simulink model "mano_buena_pinza_paper"  (R2025a)
settings: Solver=ode23  StartTime=0.0  StopTime=10.5  FixedStep=20e-3  MaxStep=1e-3  RelTol=1e-2  AbsTol=1e-4
model workspace: external: MATLAB File mano_vf_DataFile1.m (data not in the file)
undefined symbols (not defined in the file): smiData, X, Y, Z
libraries: sm_lib x268, nesl_utility x26
(part 7 of 7)

== system mano_buena_pinza_paper/Pulgar/Pulgar4/Tierra_pulgar1_RIGID ==
  ReferenceFrame : sm_lib/Frames and Transforms/Reference Frame
  Solid : sm_lib/Body Elements/File Solid  ExtGeomFileName=Tierra_pulgar_ipt_749dbfaf.STEP  UnitType=FromFile  ExtGeomFileUnits=m  StepReaderType=HEX  ExportConvexHullGeometry=on  InertiaType=Custom  BasedOnType=DensityFromFile  Density=1000  DensityUnits=kg/m^3  Mass=smiData.Solid(3).mass  MassUnits=kg  CenterOfMass=smiData.Solid(3).CoM  CenterOfMassUnits=mm  MomentsOfInertia=smiData.Solid(3).MoI  MomentsOfInertiaUnits=kg*mm^2  ProductsOfInertia=smiData.Solid(3).PoI  ProductsOfInertiaUnits=kg*mm^2  GraphicType=FromGeometry  MarkerShape=Sphere  MarkerSize=10  GraphicVisPropType=SimpleVisualProperties  GraphicDiffuseColor=smiData.Solid(3).color  GraphicOpacity=smiData.Solid(3).opacity  GraphicSpecularColor=[0.5 0.5 0.5 1.0]  GraphicAmbientColor=[0.15 0.15 0.15 1.0]  GraphicEmissiveColor=[0.0 0.0 0.0 1.0]  GraphicShininess=75  DoExposeReferenceFrame=on  SerializedFrames=<Frames/>
  Transform : sm_lib/Frames and Transforms/Rigid Transform  RotationMethod=ArbitraryAxis  FollAlignAxisA=+X  BaseAlignAxisA=+Y  FollAlignAxisB=+Y  BaseAlignAxisB=+Z  RotationStandardAxis=+Z  RotationAngle=smiData.RigidTransform(82).angle  RotationAngleUnits=rad  RotationArbitraryAxis=smiData.RigidTransform(82).axis  RotationSequenceAxes=FollowerAxes  RotationSequence=XYX  RotationSequenceAngles=[0 0 0]  RotationSequenceAnglesUnits=deg  RotationMatrix=[1 0 0;0 1 0;0 0 1]  Quaternion=[1 0 0 0]  TranslationMethod=Cartesian  TranslationCartesianOffset=smiData.RigidTransform(82).translation  TranslationCartesianOffsetUnits=mm  TranslationStandardAxis=+Z  TranslationStandardOffset=0  TranslationStandardOffsetUnits=m  TranslationROffset=0  TranslationROffsetUnits=m  TranslationThetaOffset=0  TranslationThetaOffsetUnits=deg  TranslationZOffset=0  TranslationZOffsetUnits=m
  Transform1 : sm_lib/Frames and Transforms/Rigid Transform  RotationMethod=ArbitraryAxis  FollAlignAxisA=+X  BaseAlignAxisA=+Y  FollAlignAxisB=+Y  BaseAlignAxisB=+Z  RotationStandardAxis=+Z  RotationAngle=smiData.RigidTransform(91).angle  RotationAngleUnits=rad  RotationArbitraryAxis=smiData.RigidTransform(91).axis  RotationSequenceAxes=FollowerAxes  RotationSequence=XYX  RotationSequenceAngles=[0 0 0]  RotationSequenceAnglesUnits=deg  RotationMatrix=[1 0 0;0 1 0;0 0 1]  Quaternion=[1 0 0 0]  TranslationMethod=Cartesian  TranslationCartesianOffset=smiData.RigidTransform(91).translation  TranslationCartesianOffsetUnits=mm  TranslationStandardAxis=+Z  TranslationStandardOffset=0  TranslationStandardOffsetUnits=m  TranslationROffset=0  TranslationROffsetUnits=m  TranslationThetaOffset=0  TranslationThetaOffsetUnits=deg  TranslationZOffset=0  TranslationZOffsetUnits=m
  F : PMIOPort  Side=Left
  F1 : PMIOPort  Port=2  Side=Right
  F2 : PMIOPort  Port=3  Side=Right
  connections:
  Solid/RConn1 -- ReferenceFrame/RConn1 -- Transform/LConn1 -- Transform1/LConn1
  Transform/RConn1 -- F/RConn1
  Transform1/RConn1 -- F1/RConn1
  F2/RConn1 -- Solid/LConn1

== system mano_buena_pinza_paper/Pulgar/Pulgar4/distal_pulgar1_RIGID ==
  ReferenceFrame : sm_lib/Frames and Transforms/Reference Frame
  Solid : sm_lib/Body Elements/File Solid  ExtGeomFileName=distal_pulgar_ipt_baa67ac8.STEP  UnitType=FromFile  ExtGeomFileUnits=m  StepReaderType=HEX  ExportConvexHullGeometry=on  InertiaType=Custom  BasedOnType=DensityFromFile  Density=1000  DensityUnits=kg/m^3  Mass=smiData.Solid(5).mass  MassUnits=kg  CenterOfMass=smiData.Solid(5).CoM  CenterOfMassUnits=mm  MomentsOfInertia=smiData.Solid(5).MoI  MomentsOfInertiaUnits=kg*mm^2  ProductsOfInertia=smiData.Solid(5).PoI  ProductsOfInertiaUnits=kg*mm^2  GraphicType=FromGeometry  MarkerShape=Sphere  MarkerSize=10  GraphicVisPropType=SimpleVisualProperties  GraphicDiffuseColor=smiData.Solid(5).color  GraphicOpacity=smiData.Solid(5).opacity  GraphicSpecularColor=[0.5 0.5 0.5 1.0]  GraphicAmbientColor=[0.15 0.15 0.15 1.0]  GraphicEmissiveColor=[0.0 0.0 0.0 1.0]  GraphicShininess=75  DoExposeReferenceFrame=on  SerializedFrames=<Frames/>
  Transform : sm_lib/Frames and Transforms/Rigid Transform  RotationMethod=ArbitraryAxis  FollAlignAxisA=+X  BaseAlignAxisA=+Y  FollAlignAxisB=+Y  BaseAlignAxisB=+Z  RotationStandardAxis=+Z  RotationAngle=smiData.RigidTransform(35).angle  RotationAngleUnits=rad  RotationArbitraryAxis=smiData.RigidTransform(35).axis  RotationSequenceAxes=FollowerAxes  RotationSequence=XYX  RotationSequenceAngles=[0 0 0]  RotationSequenceAnglesUnits=deg  RotationMatrix=[1 0 0;0 1 0;0 0 1]  Quaternion=[1 0 0 0]  TranslationMethod=Cartesian  TranslationCartesianOffset=smiData.RigidTransform(35).translation  TranslationCartesianOffsetUnits=mm  TranslationStandardAxis=+Z  TranslationStandardOffset=0  TranslationStandardOffsetUnits=m  TranslationROffset=0  TranslationROffsetUnits=m  TranslationThetaOffset=0  TranslationThetaOffsetUnits=deg  TranslationZOffset=0  TranslationZOffsetUnits=m
  Transform1 : sm_lib/Frames and Transforms/Rigid Transform  RotationMethod=ArbitraryAxis  FollAlignAxisA=+X  BaseAlignAxisA=+Y  FollAlignAxisB=+Y  BaseAlignAxisB=+Z  RotationStandardAxis=+Z  RotationAngle=smiData.RigidTransform(39).angle  RotationAngleUnits=rad  RotationArbitraryAxis=smiData.RigidTransform(39).axis  RotationSequenceAxes=FollowerAxes  RotationSequence=XYX  RotationSequenceAngles=[0 0 0]  RotationSequenceAnglesUnits=deg  RotationMatrix=[1 0 0;0 1 0;0 0 1]  Quaternion=[1 0 0 0]  TranslationMethod=Cartesian  TranslationCartesianOffset=smiData.RigidTransform(39).translation  TranslationCartesianOffsetUnits=mm  TranslationStandardAxis=+Z  TranslationStandardOffset=0  TranslationStandardOffsetUnits=m  TranslationROffset=0  TranslationROffsetUnits=m  TranslationThetaOffset=0  TranslationThetaOffsetUnits=deg  TranslationZOffset=0  TranslationZOffsetUnits=m
  Transform2 : sm_lib/Frames and Transforms/Rigid Transform  RotationMethod=ArbitraryAxis  FollAlignAxisA=+X  BaseAlignAxisA=+Y  FollAlignAxisB=+Y  BaseAlignAxisB=+Z  RotationStandardAxis=+Z  RotationAngle=smiData.RigidTransform(92).angle  RotationAngleUnits=rad  RotationArbitraryAxis=smiData.RigidTransform(92).axis  RotationSequenceAxes=FollowerAxes  RotationSequence=XYX  RotationSequenceAngles=[0 0 0]  RotationSequenceAnglesUnits=deg  RotationMatrix=[1 0 0;0 1 0;0 0 1]  Quaternion=[1 0 0 0]  TranslationMethod=Cartesian  TranslationCartesianOffset=smiData.RigidTransform(92).translation  TranslationCartesianOffsetUnits=mm  TranslationStandardAxis=+Z  TranslationStandardOffset=0  TranslationStandardOffsetUnits=m  TranslationROffset=0  TranslationROffsetUnits=m  TranslationThetaOffset=0  TranslationThetaOffsetUnits=deg  TranslationZOffset=0  TranslationZOffsetUnits=m
  F2 : PMIOPort  Side=Left
  F1 : PMIOPort  Port=2  Side=Right
  F : PMIOPort  Port=3  Side=Right
  F3 : PMIOPort  Port=4  Side=Left
  connections:
  Solid/RConn1 -- ReferenceFrame/RConn1 -- Transform1/LConn1 -- Transform2/LConn1 -- Transform/LConn1
  Transform/RConn1 -- F/RConn1
  Transform1/RConn1 -- F1/RConn1
  Transform2/RConn1 -- F2/RConn1
  F3/RConn1 -- Solid/LConn1

== matlab function mano_buena_pinza_paper/MATLAB Function ==
  data: tgtDeg input; refDeg output; curDeg input; refVel output
function [refDeg, refVel] = traj_block(tgtDeg, curDeg)
%#codegen
% Generador de trayectoria trapezoidal (replica traj_plan/traj_eval del main.c)
% El sample time del bloque debe ser Ts = 0.02 s (igual que el modelo discreto)

    Ts   = 0.02;
    VMAX = 40.0;     % deg/s    (TRAJ_VMAX del main.c)
    AMAX = 200.0;    % deg/s^2  (TRAJ_AMAX del main.c)

    N = numel(tgtDeg);

    persistent startDeg endDeg dirn vmax ta tc ttotal tloc active init
    if isempty(init)
        startDeg = zeros(N,1); endDeg = curDeg(:); dirn = zeros(N,1);
        vmax = zeros(N,1); ta = zeros(N,1); tc = zeros(N,1);
        ttotal = zeros(N,1); tloc = zeros(N,1); active = zeros(N,1);
        init = true;
    end

    refDeg = zeros(N,1);
    refVel = zeros(N,1);

    for i = 1:N
        % ----- Trigger de replaneo (igual que TRAJ_MOTOR) -----
        if active(i) == 0 && abs(endDeg(i)-tgtDeg(i)) > 0.05 && ...
                             abs(tgtDeg(i)-curDeg(i)) > 1.5
            D = tgtDeg(i) - curDeg(i);
            startDeg(i) = curDeg(i);
            endDeg(i)   = tgtDeg(i);
            dirn(i)     = sign(D); if dirn(i)==0, dirn(i)=1; end
            Dabs = abs(D);

            taT = VMAX / AMAX;
            da  = 0.5 * AMAX * taT^2;
            if 2*da > Dabs                 % triangular
                ta(i)   = sqrt(Dabs / AMAX);
                vmax(i) = AMAX * ta(i);
                tc(i)   = 0;
            else                            % trapezoidal
                ta(i)   = taT;
                vmax(i) = VMAX;
                tc(i)   = (Dabs - 2*da) / VMAX;
            end
            ttotal(i) = 2*ta(i) + tc(i);
            tloc(i)   = 0;
            active(i) = 1;
        end

        % ----- Evaluación del perfil (traj_eval) -----
        if active(i) == 1
            tt = tloc(i);
            if tt >= ttotal(i)
                refDeg(i) = endDeg(i); refVel(i) = 0; active(i) = 0;
            elseif tt < ta(i)                         % acelerando
                refVel(i) = dirn(i)*(AMAX*tt);
                refDeg(i) = startDeg(i) + dirn(i)*(0.5*AMAX*tt^2);
            elseif tt < ta(i)+tc(i)                   % crucero
                tcr = tt - ta(i);
                refVel(i) = dirn(i)*vmax(i);
                refDeg(i) = startDeg(i) + dirn(i)*(0.5*AMAX*ta(i)^2 + vmax(i)*tcr);
            else                                       % desacelerando
                td = tt - ta(i) - tc(i);
                refVel(i) = dirn(i)*(vmax(i) - AMAX*td);
                refDeg(i) = startDeg(i) + dirn(i)*(0.5*AMAX*ta(i)^2 + ...
                            vmax(i)*tc(i) + vmax(i)*td - 0.5*AMAX*td^2);
            end
            tloc(i) = tloc(i) + Ts;
        else
            refDeg(i) = endDeg(i); refVel(i) = 0;       % mantiene el objetivo
        end
    end
end

== matlab function mano_buena_pinza_paper/INV_CINEMATIC ==
  settings: updateMethod=DISCRETE
  data: F_indice input double size=1; F_pulgar input double size=1; F_threshold parameter double size=1; theta_real_deg input double; setpoints_deg output double size=[11 1]
function setpoints_deg = TipPinchGrasp_setpoint(F_indice, F_pulgar, F_threshold, theta_real_deg)

    % PERSISTENTES
    persistent contacted_indice contacted_pulgar theta_hold theta_grasp_calc stage theta_grasp_real

    if isempty(contacted_indice)
        contacted_indice  = false;
        contacted_pulgar  = false;
        theta_hold        = zeros(11,1);
        theta_grasp_calc  = zeros(11,1);
        stage             = 1;   % 1=ABD pulgar, 2=MCP pulgar, 3=indice+soporte
        theta_grasp_real  = [];  % objetivo de dedos recomputado con pulgar real
    end

    % ========================================================
    %  AJUSTE MANUAL - PIP del INDICE (junta 3)
    %  Suma en grados al PIP calculado por la IK.
    %    negativo  -> menos flexion  (retrae la punta, corrige sobrepaso)
    %    positivo  -> mas flexion
    %  Poner 0.0 para dejar el valor tal cual lo entrega la IK.
    % ========================================================
    pip_indice_ajuste_deg = -12.5;   % <-- AJUSTAR AQUI

    % PARAMETROS
    freeze_abd_on_contact = true;   % congelar ABD ademas del MCP al tocar el pulgar
    tol_deg               = 2.0;    % tolerancia de llegada por fase

    retroceso_mcp_pulgar_deg = 0.0;
    retroceso_dedos_deg      = 0.0;

    % Angulos objetivo iniciales (posicion de reposo)
    theta_0 = [(-143.6600000000000/-3.8151)-0.1556; ...
               -175.12670700588635+180-4.8; ...
                1.4516897910062629; ...
               -173.87060141711123+180-6.0; ...
                8.4987069032538063; ...
               -177.26207595048015+180-2.7; ...
                1.8689078585581695e-13; ...
               -177.71054335982637+180-2.1; ...
               10.54754775353744; ...
               -175.51191256300692+180-5.8; ...
               -164.83058974690246+180-14];

    % Calcular theta_grasp una sola vez
    if theta_grasp_calc(1) == 0.0 && theta_grasp_calc(2) == 0.0
        theta_grasp_calc = calcular_tip_pinch_IK(theta_0);
        fprintf('=== theta_grasp TipPinch (setpoint) ===\n');
        nombres = {'ABD_indice','MCP_indice','PIP_indice','MCP_medio','PIP_medio',...
                   'MCP_anular','PIP_anular','MCP_menique','PIP_menique','MCP_pulgar','ABD_pulgar'};
        for k = 1:11
            fprintf('  [%2d] %-14s  theta_0=%7.3f  grasp=%7.3f\n', ...
                    int32(k), nombres{k}, theta_0(k), theta_grasp_calc(k));
        end
    end
    theta_grasp = theta_grasp_calc;

    % Setpoint base: todo en reposo, salvo la junta base
    setpoints_deg    = theta_0;
    setpoints_deg(1) = theta_grasp(1);   % ABD indice, posicionada desde t=0

    % FASE 1: ABD del pulgar
    if stage >= 1
        setpoints_deg(11) = theta_grasp(11);
    end

    % Avance 1 -> 2: ABD llego dentro de tolerancia (no tiene sensor propio)
    if stage == 1
        if abs(theta_real_deg(11) - theta_grasp(11)) < tol_deg
            stage = 2;
        end
    end

    % FASE 2: MCP del pulgar
    if stage >= 2
        setpoints_deg(10) = theta_grasp(10);
    end

    % Freeze pulgar (solo en fase 2): MCP con retroceso; ABD sin retroceso
    if stage == 2 && ~contacted_pulgar && (F_pulgar > F_threshold)
        contacted_pulgar = true;
        theta_hold(10)   = theta_real_deg(10) - retroceso_mcp_pulgar_deg;
        if freeze_abd_on_contact
            theta_hold(11) = theta_real_deg(11);
        end
        % recomputar objetivos de dedos contra la yema REAL del pulgar congelado
        abd_pulgar_real = theta_grasp(11);
        if freeze_abd_on_contact
            abd_pulgar_real = theta_hold(11);
        end
        theta_grasp_real = recompute_dedos_con_pulgar_fijo( ...
                               theta_hold(10), abd_pulgar_real, theta_grasp);
    end
    if contacted_pulgar
        setpoints_deg(10) = theta_hold(10);
        if freeze_abd_on_contact
            setpoints_deg(11) = theta_hold(11);
        end
    end

    % Avance 2 -> 3: pulgar (MCP) toco o llego dentro de tolerancia
    if stage == 2
        llego_mcp_pulgar = abs(theta_real_deg(10) - theta_grasp(10)) < tol_deg;
        if contacted_pulgar || llego_mcp_pulgar
            stage = 3;
        end
    end

    % FASE 3: indice + dedos de soporte (juntas 2-9)
    if stage >= 3
        if ~isempty(theta_grasp_real)
            setpoints_deg(2:9) = theta_grasp_real(2:9);
        else
            setpoints_deg(2:9) = theta_grasp(2:9);
        end
        % AJUSTE MANUAL del PIP del indice (junta 3), aplicado a la consigna
        setpoints_deg(3) = setpoints_deg(3) + pip_indice_ajuste_deg;
    end

    % Freeze indice + soporte: latch del angulo real al tocar
    if stage >= 3 && ~contacted_indice && (F_indice > F_threshold)
        contacted_indice = true;
        theta_hold(2:9)  = theta_real_deg(2:9) - retroceso_dedos_deg;
    end
    if contacted_indice
        setpoints_deg(2:9) = theta_hold(2:9);
    end

end


% ============================================================
%  Recomputa objetivos de indice + dedos de soporte usando la
%  yema REAL del pulgar congelado, en lugar de la ideal.
% ============================================================
function theta_new = recompute_dedos_con_pulgar_fijo(mcp_pulgar_real, abd_pulgar_real, theta_grasp_ideal)
    offset_i  =  33.300; L0_i  = 27.0; L1_i  = 55.000; L2_i  = 38.160; L3_i  = 34.000;
    offset_m  =   0.000; L0_m  = 27.0; L1_m  = 69.000; L2_m  = 45.500; L3_m  = 34.800;
    offset_a  = -33.300; L0_a  = 27.0; L1_a  = 61.500; L2_a  = 38.160; L3_a  = 31.700;
    offset_me = -66.600; L0_me = 27.0; L1_me = 55.000; L2_me = 33.210; L3_me = 27.300;

    L0_p = 45.510; L1_p = 33.210; L2_p = 22.000;
    pos_base_pulgar = [26.127; -73.939; 0.0];
    tilt = 50.0;
    espesor_objeto_mm = 0.0;

    P_MCP_i = [L0_i; 0];

    [yema_real, ~] = fk_pulgar_y_jacobiano(abd_pulgar_real, mcp_pulgar_real, ...
                        pos_base_pulgar, tilt, L0_p, L1_p, L2_p);
    Y_t     = yema_real(2);
    Z_t     = yema_real(3);
    Y_t_obj = Y_t + espesor_objeto_mm;

    [MCP_i, PIP_i] = ik_dedo_2D([Y_t_obj; Z_t], P_MCP_i, L1_i, L2_i, L3_i, 1);
    [~, joints_i]  = forwardFinger(MCP_i, PIP_i, L1_i, L2_i, L3_i, P_MCP_i, 1);
    punta_indice_3D = [offset_i; joints_i(1,4); joints_i(2,4)];

    [MCP_m, PIP_m] = ik_dedo(punta_indice_3D, offset_m, L0_m, L1_m, L2_m, L3_m, 2);
    [MCP_a, PIP_a] = ik_dedo(punta_indice_3D, offset_a, L0_a, L1_a, L2_a, L3_a, 3);

    th4_ref    = DIP_from_PIP(PIP_i, 4);
    alcance_me = L0_me + L1_me*cosd(MCP_i) + L2_me*cosd(MCP_i+PIP_i) ...
                 + L3_me*cosd(MCP_i+PIP_i+th4_ref);
    r_target_me = punta_indice_3D(2);
    z_target_me = punta_indice_3D(3);
    if r_target_me > alcance_me * 0.95
        factor      = (alcance_me * 0.90) / r_target_me;
        r_target_me = r_target_me * factor;
        z_target_me = z_target_me * factor;
    end
    punta_3D_me = [offset_me; r_target_me; z_target_me];
    [MCP_me, PIP_me] = ik_dedo(punta_3D_me, offset_me, L0_me, L1_me, L2_me, L3_me, 4);

    theta_new     = theta_grasp_ideal;
    theta_new(2)  = MCP_i;   theta_new(3)  = PIP_i;
    theta_new(4)  = MCP_m;   theta_new(5)  = PIP_m;
    theta_new(6)  = MCP_a;   theta_new(7)  = PIP_a;
    theta_new(8)  = MCP_me;  theta_new(9)  = PIP_me;

    fprintf(['[TipPinch] Recompute con pulgar real: MCP_p=%.2f ABD_p=%.2f ', ...
             '-> yema real Y=%.2f Z=%.2f | MCP_i=%.2f PIP_i=%.2f\n'], ...
            mcp_pulgar_real, abd_pulgar_real, Y_t, Z_t, MCP_i, PIP_i);
end


% ============================================================
%  Calcula angulos objetivo por interseccion en el plano X
% ============================================================
function theta_grasp = calcular_tip_pinch_IK(theta_0)
    offset_i  =  33.300; L0_i  = 27.0; L1_i  = 55.000; L2_i  = 38.160; L3_i  = 34.000;
    offset_m  =   0.000; L0_m  = 27.0; L1_m  = 69.000; L2_m  = 45.500; L3_m  = 34.800;
    offset_a  = -33.300; L0_a  = 27.0; L1_a  = 61.500; L2_a  = 38.160; L3_a  = 31.700;
    offset_me = -66.600; L0_me = 27.0; L1_me = 55.000; L2_me = 33.210; L3_me = 27.300;

    L0_p = 45.510;
    L1_p = 33.210;
    L2_p = 22.000;
    pos_base_pulgar = [26.127; -73.939; 0.0];
    tilt = 50.0;
    X_objetivo_plano = offset_i;
    P_MCP_i = [L0_i; 0];

    mcp_candidatos = 0.0:1.0:80.0;
    gap_tol        = 1.0;
    espesor_objeto_mm = 20.0;

    best_Z      = -inf;
    sel_mcp     = 20.0;  sel_abd   = 15.0;
    sel_MCP_i   = 0.0;   sel_PIP_i = 0.0;
    sel_yema    = [offset_i; 0; 0];
    sel_gap     = inf;
    hay_conv    = false;

    best_cost   = inf;
    fb_mcp      = 20.0;  fb_abd    = 15.0;
    fb_MCP_i    = 0.0;   fb_PIP_i  = 0.0;
    fb_yema     = [offset_i; 0; 0];
    encontrado  = false;

    for mcp_try = mcp_candidatos
        [abd_try, yema_try] = buscar_abd_pulgar_en_plano(...
            X_objetivo_plano, mcp_try, pos_base_pulgar, tilt, L0_p, L1_p, L2_p);

        if abs(yema_try(1) - X_objetivo_plano) > 1.0
            continue;
        end

        Y_t = yema_try(2);
        Z_t = yema_try(3);
        Y_t_obj = Y_t + espesor_objeto_mm;

        [MCP_try, PIP_try] = ik_dedo_2D([Y_t_obj; Z_t], P_MCP_i, L1_i, L2_i, L3_i, 1);
        [p_tip_i, ~]       = forwardFinger(MCP_try, PIP_try, L1_i, L2_i, L3_i, P_MCP_i, 1);

        residual = norm([Y_t_obj; Z_t] - p_tip_i);

        if residual < best_cost
            best_cost  = residual;
            fb_mcp     = mcp_try;   fb_abd   = abd_try;
            fb_MCP_i   = MCP_try;   fb_PIP_i = PIP_try;
            fb_yema    = yema_try;
            encontrado = true;
        end

        if residual < gap_tol && Z_t > best_Z
            best_Z    = Z_t;
            sel_mcp   = mcp_try;    sel_abd   = abd_try;
            sel_MCP_i = MCP_try;    sel_PIP_i = PIP_try;
            sel_yema  = yema_try;
            sel_gap   = residual;
            hay_conv  = true;
        end
    end

    if hay_conv
        best_mcp   = sel_mcp;   best_abd   = sel_abd;
        best_MCP_i = sel_MCP_i; best_PIP_i = sel_PIP_i;
        best_yema  = sel_yema;
        best_cost  = sel_gap;
    elseif encontrado
        warning('[TipPinch] Ninguna postura converge bajo gap_tol=%.2f mm. Usando la de menor gap (%.3f mm).', ...
                gap_tol, best_cost);
        best_mcp   = fb_mcp;    best_abd   = fb_abd;
        best_MCP_i = fb_MCP_i;  best_PIP_i = fb_PIP_i;
        best_yema  = fb_yema;
    else
        error('[TipPinch] El pulgar no pudo alcanzar el plano X = %.1f en ningun MCP del barrido.', X_objetivo_plano);
    end

    mcp_pulgar  = best_mcp;
    ip_pulgar   = DIP_from_PIP(mcp_pulgar, 5);
    abd_pulgar  = best_abd;
    MCP_i       = best_MCP_i;
    PIP_i       = best_PIP_i;
    Y_encuentro = best_yema(2);
    Z_encuentro = best_yema(3);

    [~, joints_i]   = forwardFinger(MCP_i, PIP_i, L1_i, L2_i, L3_i, P_MCP_i, 1);
    punta_indice_3D = [offset_i; joints_i(1,4); joints_i(2,4)];

    fprintf('[TipPinch] Encuentro: MCP_pulgar=%.1f deg  (IP_acoplado=%.1f deg)  ABD_pulgar=%.2f deg  gap=%.3f mm\n', ...
            mcp_pulgar, ip_pulgar, abd_pulgar, best_cost);
    fprintf('[TipPinch] Punto de encuentro (mas alejado en +z): Y=%.2f mm  Z=%.2f mm\n', ...
            Y_encuentro, Z_encuentro);

    [MCP_m, PIP_m] = ik_dedo(punta_indice_3D, offset_m, L0_m, L1_m, L2_m, L3_m, 2);
    [MCP_a, PIP_a] = ik_dedo(punta_indice_3D, offset_a, L0_a, L1_a, L2_a, L3_a, 3);

    th4_ref    = DIP_from_PIP(PIP_i, 4);
    alcance_me = L0_me + L1_me * cosd(MCP_i) + L2_me * cosd(MCP_i + PIP_i) + L3_me * cosd(MCP_i + PIP_i + th4_ref);
    r_target_me = punta_indice_3D(2);
    z_target_me = punta_indice_3D(3);
    if r_target_me > alcance_me * 0.95
        factor      = (alcance_me * 0.90) / r_target_me;
        r_target_me = r_target_me * factor;
        z_target_me = z_target_me * factor;
    end
    punta_3D_me = [offset_me; r_target_me; z_target_me];
    [MCP_me, PIP_me] = ik_dedo(punta_3D_me, offset_me, L0_me, L1_me, L2_me, L3_me, 4);

    theta_grasp     = theta_0;
    theta_grasp(2)  = MCP_i;
    theta_grasp(3)  = PIP_i;
    theta_grasp(4)  = MCP_m;
    theta_grasp(5)  = PIP_m;
    theta_grasp(6)  = MCP_a;
    theta_grasp(7)  = PIP_a;
    theta_grasp(8)  = MCP_me;
    theta_grasp(9)  = PIP_me;
    theta_grasp(10) = mcp_pulgar;
    theta_grasp(11) = abd_pulgar;
    fprintf('[Tip Pinch] Interseccion lograda en X = 33.3 mm\n');
    fprintf('            Coordenadas de contacto reales: Y = %.2f mm, Z = %.2f mm\n', Y_encuentro, Z_encuentro);
end


% ============================================================
%  Buscador numerico de abduccion del pulgar para plano fijo X
% ============================================================
function [abd_out, yema_3D] = buscar_abd_pulgar_en_plano(X_target, ip_fijo, pos_base, tilt, L0, L1, L2)
    abd = 15.0;
    max_iter = 200;
    tol = 0.05;
    learning_rate = 0.5;

    for iter = 1:max_iter
        [yema, J] = fk_pulgar_y_jacobiano(abd, ip_fijo, pos_base, tilt, L0, L1, L2);
        error_x = X_target - yema(1);

        if abs(error_x) < tol
            break;
        end

        if abs(J(1,1)) > 1e-4
            abd = abd + learning_rate * (error_x / J(1,1));
        else
            abd = abd + learning_rate * sign(error_x);
        end

        abd = max(0.0, min(60.0, abd));
    end

    [yema_3D, ~] = fk_pulgar_y_jacobiano(abd, ip_fijo, pos_base, tilt, L0, L1, L2);
    abd_out = abd;
end


% ============================================================
%  FK del pulgar + Jacobiano
% ============================================================
function [yema_3D, J] = fk_pulgar_y_jacobiano(abd, ip, pos_base, tilt, L0, L1, L2)

    k = pi / 180.0;

    Yl = [ cosd(tilt);  sind(tilt); 0];
    Xl = [ sind(tilt); -cosd(tilt); 0];
    Zl = cross(Xl, Yl);  Zl = Zl / norm(Zl);
    R  = [Xl, Yl, Zl];

    th3      = DIP_from_PIP(ip, 5);
    dth3_dip = dDIP_dPIP(ip, 5);

    c1   = cosd(abd);
    s1   = sind(abd);

    r2d = L0 + L1*cosd(ip) + L2*cosd(ip + th3);
    h2d =      L1*sind(ip) + L2*sind(ip + th3);

    yema_loc = [-h2d; c1*r2d; s1*r2d];
    yema_3D  = pos_base + R * yema_loc;

    dr_dip = k * (-L1*sind(ip) - L2*sind(ip + th3)*(1 + dth3_dip));
    dh_dip = k * ( L1*cosd(ip) + L2*cosd(ip + th3)*(1 + dth3_dip));

    dloc_dabd = k * [ 0; -s1*r2d; c1*r2d];
    dloc_dip  =     [-dh_dip; c1*dr_dip; s1*dr_dip];

    J = R * [dloc_dabd, dloc_dip];

end


% ============================================================
%  IK 2D (Levenberg-Marquardt)
% ============================================================
function [th2_out, th3_out] = ik_dedo_2D(target_2d, P_MCP, L1, L2, L3, dedo_id)
    th2 = 20.0;
    th3 = 20.0;
    lambda    = 0.01;
    max_iter  = 300;
    tol       = 0.15;
    for iter = 1:max_iter
        [p_tip, ~] = forwardFinger(th2, th3, L1, L2, L3, P_MCP, dedo_id);
        e = target_2d - p_tip;
        if norm(e) < tol
            break;
        end
        J   = jacobianFinger(th2, th3, L1, L2, L3, dedo_id);
        dth = (J'*J + lambda^2 * eye(2)) \ (J' * e);
        th2 = max(0.0, min(90.0, th2 + dth(1)));
        th3 = max(0.0, min(90.0, th3 + dth(2)));
    end
    th2_out = max(0.0, min(90.0, th2));
    th3_out = max(0.0, min(90.0, th3));
end


% ============================================================
%  IK dedo (wrapper 3D -> 2D sagital)
% ============================================================
function [th2_out, th3_out] = ik_dedo(punta_3D, ~, L0, L1, L2, L3, dedo_id)
    target_2d = [punta_3D(2); punta_3D(3)];
    P_MCP     = [L0; 0];
    [th2_out, th3_out] = ik_dedo_2D(target_2d, P_MCP, L1, L2, L3, dedo_id);
end


% ============================================================
%  FK 2D
% ============================================================
function [p_tip, joints] = forwardFinger(th2, th3, L1, L2, L3, P_MCP, dedo_id)
    th4    = DIP_from_PIP(th3, dedo_id);
    R2     = rot2d(th2);
    R3     = rot2d(th2 + th3);
    R4     = rot2d(th2 + th3 + th4);
    P1     = P_MCP;
    P2     = P1 + R2 * [L1; 0];
    P3     = P2 + R3 * [L2; 0];
    P4     = P3 + R4 * [L3; 0];
    p_tip  = P4;
    joints = [P1 P2 P3 P4];
end


% ============================================================
%  Jacobiano 2D
% ============================================================
function J = jacobianFinger(th2, th3, L1, L2, L3, dedo_id)
    k          = pi / 180.0;
    th4        = DIP_from_PIP(th3, dedo_id);
    dth4_dth3  = dDIP_dPIP(th3, dedo_id);
    phi2r      = deg2rad(th2);
    phi3r      = deg2rad(th2 + th3);
    phi4r      = deg2rad(th2 + th3 + th4);
    dphi4_dth3 = 1.0 + dth4_dth3;

    dr_dth2 = k * (-sin(phi2r)*L1 - sin(phi3r)*L2 - sin(phi4r)*L3);
    dz_dth2 = k * ( cos(phi2r)*L1 + cos(phi3r)*L2 + cos(phi4r)*L3);
    dr_dth3 = k * (-sin(phi3r)*L2 - sin(phi4r)*dphi4_dth3*L3);
    dz_dth3 = k * ( cos(phi3r)*L2 + cos(phi4r)*dphi4_dth3*L3);
    J = [dr_dth2 dr_dth3; dz_dth2 dz_dth3];
end


% ============================================================
%  DIP acoplado al PIP (casos 1-4 = dedos largos, caso 5 = pulgar)
% ============================================================
function th4 = DIP_from_PIP(th3, dedo_id)
    if dedo_id == 1
        th4 = (-0.00000016)*th3^4 + (0.00006721)*th3^3 ...
            + (-0.01062799)*th3^2 + (1.68304757)*th3 + (0.04984945);
    elseif dedo_id == 2
        th4 = (0.00000107)*th3^4  + (-0.00012334)*th3^3 ...
            + (0.00087773)*th3^2  + (1.33867879)*th3  + (0.21523916);
    elseif dedo_id == 3
        th4 = (-0.00000020)*th3^4 + (0.00007387)*th3^3 ...
            + (-0.01090612)*th3^2 + (1.68680914)*th3  + (0.04021311);
    elseif dedo_id == 4
        th4 = (-0.00000010)*th3^4 + (0.00005985)*th3^3 ...
            + (-0.01029053)*th3^2 + (1.67216440)*th3  + (0.04004136);
    elseif dedo_id == 5 % PULGAR
        th4 = (0.00000075)*th3^4  + (-0.00008762)*th3^3 ...
            + (0.00106596)*th3^2  + (1.27148703)*th3  + (0.14418172);
    else
        th4 = 0.0;
    end
    th4 = max(0.0, min(90.0, th4));
end


% ============================================================
%  Derivada DIP respecto al PIP (casos 1-4 + caso 5 = pulgar)
% ============================================================
function dth4 = dDIP_dPIP(th3, dedo_id)
    if dedo_id == 1
        dth4 = 4*(-0.00000016)*th3^3 + 3*(0.00006721)*th3^2 ...
             + 2*(-0.01062799)*th3   + (1.68304757);
    elseif dedo_id == 2
        dth4 = 4*(0.00000107)*th3^3  + 3*(-0.00012334)*th3^2 ...
             + 2*(0.00087773)*th3    + (1.33867879);
    elseif dedo_id == 3
        dth4 = 4*(-0.00000020)*th3^3 + 3*(0.00007387)*th3^2 ...
             + 2*(-0.01090612)*th3   + (1.68680914);
    elseif dedo_id == 4
        dth4 = 4*(-0.00000010)*th3^3 + 3*(0.00005985)*th3^2 ...
             + 2*(-0.01029053)*th3   + (1.67216440);
    elseif dedo_id == 5 % PULGAR
        dth4 = 4*(0.00000075)*th3^3  + 3*(-0.00008762)*th3^2 ...
             + 2*(0.00106596)*th3    + (1.27148703);
    else
        dth4 = 0.0;
    end
end


% ============================================================
%  Rotacion 2D
% ============================================================
function R = rot2d(th)
    R = [cosd(th) -sind(th); sind(th) cosd(th)];
end

== matlab function mano_buena_pinza_paper/MATLAB Function1 ==
  data: tgtDeg input; refDeg output; curDeg input; refVel output
function [refDeg, refVel] = traj_block(tgtDeg, curDeg)
%#codegen
% Generador de trayectoria trapezoidal (replica traj_plan/traj_eval del main.c)
% El sample time del bloque debe ser Ts = 0.02 s (igual que el modelo discreto)

    Ts   = 0.02;
    VMAX = 40.0;     % deg/s    (TRAJ_VMAX del main.c)
    AMAX = 200.0;    % deg/s^2  (TRAJ_AMAX del main.c)

    N = numel(tgtDeg);

    persistent startDeg endDeg dirn vmax ta tc ttotal tloc active init
    if isempty(init)
        startDeg = zeros(N,1); endDeg = curDeg(:); dirn = zeros(N,1);
        vmax = zeros(N,1); ta = zeros(N,1); tc = zeros(N,1);
        ttotal = zeros(N,1); tloc = zeros(N,1); active = zeros(N,1);
        init = true;
    end

    refDeg = zeros(N,1);
    refVel = zeros(N,1);

    for i = 1:N
        % ----- Trigger de replaneo (igual que TRAJ_MOTOR) -----
        if active(i) == 0 && abs(endDeg(i)-tgtDeg(i)) > 0.05 && ...
                             abs(tgtDeg(i)-curDeg(i)) > 1.5
            D = tgtDeg(i) - curDeg(i);
            startDeg(i) = curDeg(i);
            endDeg(i)   = tgtDeg(i);
            dirn(i)     = sign(D); if dirn(i)==0, dirn(i)=1; end
            Dabs = abs(D);

            taT = VMAX / AMAX;
            da  = 0.5 * AMAX * taT^2;
            if 2*da > Dabs                 % triangular
                ta(i)   = sqrt(Dabs / AMAX);
                vmax(i) = AMAX * ta(i);
                tc(i)   = 0;
            else                            % trapezoidal
                ta(i)   = taT;
                vmax(i) = VMAX;
                tc(i)   = (Dabs - 2*da) / VMAX;
            end
            ttotal(i) = 2*ta(i) + tc(i);
            tloc(i)   = 0;
            active(i) = 1;
        end

        % ----- Evaluación del perfil (traj_eval) -----
        if active(i) == 1
            tt = tloc(i);
            if tt >= ttotal(i)
                refDeg(i) = endDeg(i); refVel(i) = 0; active(i) = 0;
            elseif tt < ta(i)                         % acelerando
                refVel(i) = dirn(i)*(AMAX*tt);
                refDeg(i) = startDeg(i) + dirn(i)*(0.5*AMAX*tt^2);
            elseif tt < ta(i)+tc(i)                   % crucero
                tcr = tt - ta(i);
                refVel(i) = dirn(i)*vmax(i);
                refDeg(i) = startDeg(i) + dirn(i)*(0.5*AMAX*ta(i)^2 + vmax(i)*tcr);
            else                                       % desacelerando
                td = tt - ta(i) - tc(i);
                refVel(i) = dirn(i)*(vmax(i) - AMAX*td);
                refDeg(i) = startDeg(i) + dirn(i)*(0.5*AMAX*ta(i)^2 + ...
                            vmax(i)*tc(i) + vmax(i)*td - 0.5*AMAX*td^2);
            end
            tloc(i) = tloc(i) + Ts;
        else
            refDeg(i) = endDeg(i); refVel(i) = 0;       % mantiene el objetivo
        end
    end
end

== matlab function mano_buena_pinza_paper/MATLAB Function2 ==
  data: tgtDeg input; refDeg output; curDeg input; refVel output
function [refDeg, refVel] = traj_block(tgtDeg, curDeg)
%#codegen
% Generador de trayectoria trapezoidal (replica traj_plan/traj_eval del main.c)
% El sample time del bloque debe ser Ts = 0.02 s (igual que el modelo discreto)

    Ts   = 0.02;
    VMAX = 40.0;     % deg/s    (TRAJ_VMAX del main.c)
    AMAX = 200.0;    % deg/s^2  (TRAJ_AMAX del main.c)

    N = numel(tgtDeg);

    persistent startDeg endDeg dirn vmax ta tc ttotal tloc active init
    if isempty(init)
        startDeg = zeros(N,1); endDeg = curDeg(:); dirn = zeros(N,1);
        vmax = zeros(N,1); ta = zeros(N,1); tc = zeros(N,1);
        ttotal = zeros(N,1); tloc = zeros(N,1); active = zeros(N,1);
        init = true;
    end

    refDeg = zeros(N,1);
    refVel = zeros(N,1);

    for i = 1:N
        % ----- Trigger de replaneo (igual que TRAJ_MOTOR) -----
        if active(i) == 0 && abs(endDeg(i)-tgtDeg(i)) > 0.05 && ...
                             abs(tgtDeg(i)-curDeg(i)) > 1.5
            D = tgtDeg(i) - curDeg(i);
            startDeg(i) = curDeg(i);
            endDeg(i)   = tgtDeg(i);
            dirn(i)     = sign(D); if dirn(i)==0, dirn(i)=1; end
            Dabs = abs(D);

            taT = VMAX / AMAX;
            da  = 0.5 * AMAX * taT^2;
            if 2*da > Dabs                 % triangular
                ta(i)   = sqrt(Dabs / AMAX);
                vmax(i) = AMAX * ta(i);
                tc(i)   = 0;
            else                            % trapezoidal
                ta(i)   = taT;
                vmax(i) = VMAX;
                tc(i)   = (Dabs - 2*da) / VMAX;
            end
            ttotal(i) = 2*ta(i) + tc(i);
            tloc(i)   = 0;
            active(i) = 1;
        end

        % ----- Evaluación del perfil (traj_eval) -----
        if active(i) == 1
            tt = tloc(i);
            if tt >= ttotal(i)
                refDeg(i) = endDeg(i); refVel(i) = 0; active(i) = 0;
            elseif tt < ta(i)                         % acelerando
                refVel(i) = dirn(i)*(AMAX*tt);
                refDeg(i) = startDeg(i) + dirn(i)*(0.5*AMAX*tt^2);
            elseif tt < ta(i)+tc(i)                   % crucero
                tcr = tt - ta(i);
                refVel(i) = dirn(i)*vmax(i);
                refDeg(i) = startDeg(i) + dirn(i)*(0.5*AMAX*ta(i)^2 + vmax(i)*tcr);
            else                                       % desacelerando
                td = tt - ta(i) - tc(i);
                refVel(i) = dirn(i)*(vmax(i) - AMAX*td);
                refDeg(i) = startDeg(i) + dirn(i)*(0.5*AMAX*ta(i)^2 + ...
                            vmax(i)*tc(i) + vmax(i)*td - 0.5*AMAX*td^2);
            end
            tloc(i) = tloc(i) + Ts;
        else
            refDeg(i) = endDeg(i); refVel(i) = 0;       % mantiene el objetivo
        end
    end
end

== matlab function mano_buena_pinza_paper/MATLAB Function3 ==
  data: tgtDeg input; refDeg output; curDeg input; refVel output
function [refDeg, refVel] = traj_block(tgtDeg, curDeg)
%#codegen
% Generador de trayectoria trapezoidal (replica traj_plan/traj_eval del main.c)
% El sample time del bloque debe ser Ts = 0.02 s (igual que el modelo discreto)

    Ts   = 0.02;
    VMAX = 40.0;     % deg/s    (TRAJ_VMAX del main.c)
    AMAX = 200.0;    % deg/s^2  (TRAJ_AMAX del main.c)

    N = numel(tgtDeg);

    persistent startDeg endDeg dirn vmax ta tc ttotal tloc active init
    if isempty(init)
        startDeg = zeros(N,1); endDeg = curDeg(:); dirn = zeros(N,1);
        vmax = zeros(N,1); ta = zeros(N,1); tc = zeros(N,1);
        ttotal = zeros(N,1); tloc = zeros(N,1); active = zeros(N,1);
        init = true;
    end

    refDeg = zeros(N,1);
    refVel = zeros(N,1);

    for i = 1:N
        % ----- Trigger de replaneo (igual que TRAJ_MOTOR) -----
        if active(i) == 0 && abs(endDeg(i)-tgtDeg(i)) > 0.05 && ...
                             abs(tgtDeg(i)-curDeg(i)) > 1.5
            D = tgtDeg(i) - curDeg(i);
            startDeg(i) = curDeg(i);
            endDeg(i)   = tgtDeg(i);
            dirn(i)     = sign(D); if dirn(i)==0, dirn(i)=1; end
            Dabs = abs(D);

            taT = VMAX / AMAX;
            da  = 0.5 * AMAX * taT^2;
            if 2*da > Dabs                 % triangular
                ta(i)   = sqrt(Dabs / AMAX);
                vmax(i) = AMAX * ta(i);
                tc(i)   = 0;
            else                            % trapezoidal
                ta(i)   = taT;
                vmax(i) = VMAX;
                tc(i)   = (Dabs - 2*da) / VMAX;
            end
            ttotal(i) = 2*ta(i) + tc(i);
            tloc(i)   = 0;
            active(i) = 1;
        end

        % ----- Evaluación del perfil (traj_eval) -----
        if active(i) == 1
            tt = tloc(i);
            if tt >= ttotal(i)
                refDeg(i) = endDeg(i); refVel(i) = 0; active(i) = 0;
            elseif tt < ta(i)                         % acelerando
                refVel(i) = dirn(i)*(AMAX*tt);
                refDeg(i) = startDeg(i) + dirn(i)*(0.5*AMAX*tt^2);
            elseif tt < ta(i)+tc(i)                   % crucero
                tcr = tt - ta(i);
                refVel(i) = dirn(i)*vmax(i);
                refDeg(i) = startDeg(i) + dirn(i)*(0.5*AMAX*ta(i)^2 + vmax(i)*tcr);
            else                                       % desacelerando
                td = tt - ta(i) - tc(i);
                refVel(i) = dirn(i)*(vmax(i) - AMAX*td);
                refDeg(i) = startDeg(i) + dirn(i)*(0.5*AMAX*ta(i)^2 + ...
                            vmax(i)*tc(i) + vmax(i)*td - 0.5*AMAX*td^2);
            end
            tloc(i) = tloc(i) + Ts;
        else
            refDeg(i) = endDeg(i); refVel(i) = 0;       % mantiene el objetivo
        end
    end
end
